simulink library "mobileRoboticsLib"  (R2022b)
settings: Solver=VariableStepAuto  StartTime=0.0  StopTime=10.0  RelTol=1e-3
undefined symbols (not defined in the file or in its folder): DiscIntNeverNeededParam, X, Y, Z
libraries: sm_lib x67, nesl_utility x25, $bdroot x12
(part 1 of 4)
settings Model: Creator=scastro  LastModifiedBy=mejiasal
settings SolverCC: AlgebraicLoopSolver=TrustRegion
settings DataIOCC: ReturnWorkspaceOutputs=off
settings DebuggingCC: UnconnectedInputMsg=warning  UnconnectedOutputMsg=warning  UnconnectedLineMsg=warning  SFMachineParentedDataDiag=warning  ArithmeticOperatorsInVariantConditions=warning
settings ModelReferenceCC: EnableRefExpFcnMdlSchedulingChecks=on
settings SFSimCC: SimUseLocalCustomCode=off  CustomCodeUndefinedFunction=UseInterfaceOnly
settings RTWCC: RTWUseLocalCustomCode=off

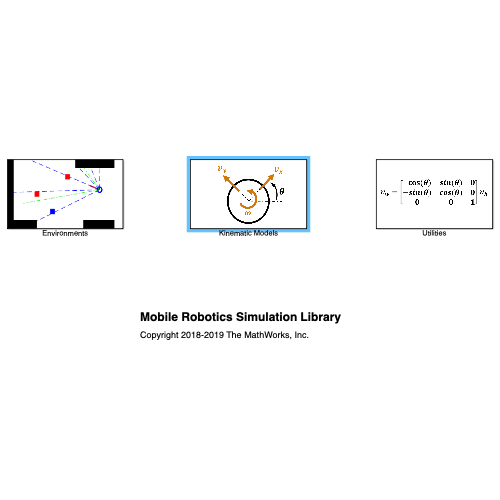
[thumbnail: Simulink's stored preview of the top-level diagram]
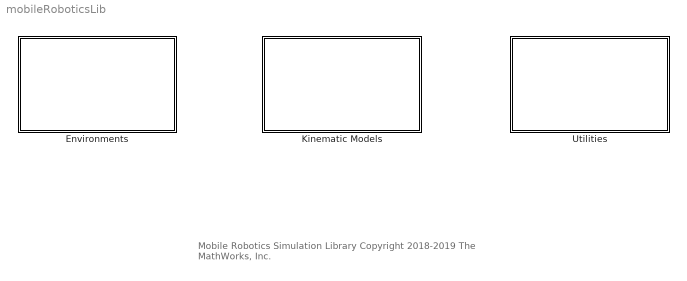
== system mobileRoboticsLib ==
  note: Mobile Robotics Simulation Library
      |
      | Copyright 2018-2019 The MathWorks, Inc.
  Environments : Subsystem
      mask Display: image('environments.PNG');
  Kinematic Models : Subsystem
      mask Display: image('kinematics.PNG')
  Utilities : Subsystem
      mask Display: image('mrsUtils.PNG');

== system mobileRoboticsLib/Environments ==
  Lidar Sensor : MATLABSystem  System=LidarSensor  sensorOffset=[ 0, 0 ]  scanAngles=[ -pi/4, 0, pi/4 ]  maxRange=5
      mask Type: LidarSensor
      mask Display:
      | disp(['Lidar' char(10) 'Sensor']);
      | port_label('input',1,'pose');
      | port_label('output',1,'ranges');
  Multi-Robot Environment : Subsystem  InitFcn=clear multiRobotVizWorld;  mask(Multi-Robot Environment){numRobots=3, mapName=, showWaypoints=off, showObjects=off, objectColors=[ 1, 0, 0; 0, 1, 0; 0, 0, 1 ], objectMarkers='s', showRobotIds=on, plotSensorLines=on}
      mask prompts: numRobots "Number of Robots"; mapName "Map Name"; showWaypoints "Accept Waypoints"; showObjects "Accept Objects"; objectColors "Object Colors"; objectMarkers "Object Markers"; showRobotIds "Show Robot IDs"; plotSensorLines "Plot Sensor Lines"
      mask help:
      | Displays map, waypoint, and object data for a multi-robot simulation.
      |
      | Use "Multi-Robot Visualizer" blocks to display individual robots in this environment.
      mask init:
      | % Configure visual tags
      | visualSub = [gcb '/Visuals'];
      | radiusBlocks = find_system(visualSub,'FollowLinks','on','LookUnderMasks','on','BlockType','From');
      | for idx = 1:numel(radiusBlocks)
      |     lh = get_param(radiusBlocks{idx},'LineHandles');
      |     delete_line(lh.Outport);
      | end
      | delete_block(radiusBlocks);
      | vecBlock = [visualSub '/Vector Concatenate'];
      | set_param(vecBlock,'NumInputs',num2str(numRobots));
      | for idx = 1:numRobots
      |     blkName = [visualSub '/From' num2str(idx)];
      |     blkPos = [0 30 200 50] + (idx-1)*[0 30 0 30];
      |     add_block('simulink/Signal Routing/From',blkName);
      |     set_param(blkName,'GotoTag',['slMultiRobotEnv_Visuals_' num2str(idx)]);
      |     set_param(blkName,'Position',blkPos);
      |     add_line(visualSub,['From' num2str(idx) '/1'],['Vector Concatenate/' num2str(idx)]);
      | end
      | 
      | % Configure pose tags
      | poseSub = [gcb '/Poses'];
      | poseBlocks = find_system(poseSub,'FollowLinks','on','LookUnderMasks','on','BlockType','From');
      | for idx = 1:numel(poseBlocks)
      |     lh = get_param(poseBlocks{idx},'LineHandles');
      |     delete_line(lh.Outport);
      | end
      | delete_block(poseBlocks);
      | vecBlock = [poseSub '/Vector Concatenate'];
      | set_param(vecBlock,'NumInputs',num2str(numRobots));
      | for idx = 1:numRobots
      |     blkName = [poseSub '/From' num2str(idx)];
      |     blkPos = [0 30 200 50] + (idx-1)*[0 30 0 30];
      |     add_block('simulink/Signal Routing/From',blkName);
      |     set_param(blkName,'GotoTag',['slMultiRobotEnv_Pose_' num2str(idx)]);
      |     set_param(blkName,'Position',blkPos);
      |     add_line(poseSub,['From' num2str(idx) '/1'],['Vector Concatenate/' num2str(idx)]);
      | end
      | 
      | % Configure range tags
      | rangeSub = [gcb '/Ranges'];
      | rangeBlocks = find_system(rangeSub,'FollowLinks','on','LookUnderMasks','on','BlockType','From');
      | for idx = 1:numel(rangeBlocks)
      |     lh = get_param(rangeBlocks{idx},'LineHandles');
      |     delete_line(lh.Outport);
      | end
      | delete_block(rangeBlocks);
      | vecBlock = [rangeSub '/Vector Concatenate'];
      | set_param(vecBlock,'NumInputs',num2str(numRobots));
      | for idx = 1:numRobots
      |     blkName = [rangeSub '/From' num2str(idx)];
      |     blkPos = [0 30 200 50] + (idx-1)*[0 30 0 30];
      |     add_block('simulink/Signal Routing/From',blkName);
      |     set_param(blkName,'GotoTag',['slMultiRobotEnv_Ranges_' num2str(idx)]);
      |     set_param(blkName,'Position',blkPos);
      |     add_line(rangeSub,['From' num2str(idx) '/1'],['Vector Concatenate/' num2str(idx)]);
      | end
      | 
      | % Initialize range sensor bus
      | internal.createRangeSensorBus;
      | 
      | % Configure object detector tags
      | objDetSub = [gcb '/ObjectDetectorParams'];
      | objDetBlocks = find_system(objDetSub,'FollowLinks','on','LookUnderMasks','on','BlockType','From');
      | for idx = 1:numel(objDetBlocks)
      |     lh = get_param(objDetBlocks{idx},'LineHandles');
      |     delete_line(lh.Outport);
      | end
      | delete_block(objDetBlocks);
      | vecBlock = [objDetSub '/Vector Concatenate'];
      | set_param(vecBlock,'NumInputs',num2str(numRobots));
      | for idx = 1:numRobots
      |     blkName = [objDetSub '/From' num2str(idx)];
      |     blkPos = [0 30 200 50] + (idx-1)*[0 30 0 30];
      |     add_block('simulink/Signal Routing/From',blkName);
      |     set_param(blkName,'GotoTag',['slMultiRobotEnv_ObjDet_' num2str(idx)]);
      |     set_param(blkName,'Position',blkPos);
      |     add_line(objDetSub,['From' num2str(idx) '/1'],['Vector Concatenate/' num2str(idx)]);
      | end
      | 
      | % Configure robot detector tags
      | robotDetSub = [gcb '/RobotDetectorParams'];
      | robotDetBlocks = find_system(robotDetSub,'FollowLinks','on','LookUnderMasks','on','BlockType','From');
      | for idx = 1:numel(robotDetBlocks)
      |     lh = get_param(robotDetBlocks{idx},'LineHandles');
      |     delete_line(lh.Outport);
      | end
      | delete_block(robotDetBlocks);
      | vecBlock = [robotDetSub '/Vector Concatenate'];
      | set_param(vecBlock,'NumInputs',num2str(numRobots));
      | for idx = 1:numRobots
      |     blkName = [robotDetSub '/From' num2str(idx)];
      |     blkPos = [0 30 200 50] + (idx-1)*[0 30 0 30];
      |     add_block('simulink/Signal Routing/From',blkName);
      |     set_param(blkName,'GotoTag',['slMultiRobotEnv_RobotDet_' num2str(idx)]);
      |     set_param(blkName,'Position',blkPos);
      |     add_line(robotDetSub,['From' num2str(idx) '/1'],['Vector Concatenate/' num2str(idx)]);
      | end
      | 
      | % Configure waypoints port
      | hasWaypointPort = ~isempty(find_system(gcb,'FollowLinks','on','LookUnderMasks','on','BlockType','Inport','Name','waypoints'));
      | if ~showWaypoints & hasWaypointPort
      |     replace_block(gcb,'FollowLinks','on','Name','waypoints','built-in/Ground','noprompt');
      | elseif showWaypoints & ~hasWaypointPort
      |     replace_block(gcb,'FollowLinks','on','Name','waypoints','built-in/Inport','noprompt'); 
      | end
      |  
      | % Configure objects port
      | hasObjectPort = ~isempty(find_system(gcb,'FollowLinks','on','LookUnderMasks','on','BlockType','Inport','Name','objects'));
      | if ~showObjects & hasObjectPort
      |     replace_block(gcb,'FollowLinks','on','Name','objects','built-in/Ground','noprompt');
      | elseif showObjects & ~hasObjectPort
      |     replace_block(gcb,'FollowLinks','on','Name','objects','built-in/Inport','noprompt');  
      | end
      | 
      | % Ensure the waypoints and objects ports are organized correctly
      | if strcmp(get_param([gcb '/waypoints'],'BlockType'),'Inport')
      |     set_param([gcb '/waypoints'],'Port','1');
      | end
      mask Help: web('matlab: edit mrsDocMultiRobotEnv')
      mask Callback showObjects:
      | mask = Simulink.Mask.get(gcb);
      | showObjects = get_param(gcb,'showObjects');
      | 
      | % Enable and disable parameters
      | indices = [find(strcmp({mask.Parameters.Name},'objectColors'));
      |            find(strcmp({mask.Parameters.Name},'objectMarkers'))];
      | 
      | for idx = 1:numel(indices)
      |     mask.Parameters(indices(idx)).Visible = showObjects;
      | end
      mask Display: fprintf('Multi-Robot\nEnvironment')
  Multi-Robot Lidar Sensor : Subsystem  mask(Multi-Robot Lidar Sensor){robotIdx=1, mapName=, sensorOffset=[0,0], scanAngles=[-pi/4 0 pi/4], maxRange=5}
      mask prompts: robotIdx "Robot Index"; mapName "Map Name"; sensorOffset "Sensor offset (x,y) [m]"; scanAngles "Scan angles [rad]"; maxRange "Maximum Range [m]"
      mask help: 2D lidar sensor simulation for multi-robot environment.
      mask init:
      | % Find number of robots 
      | mrEnvBlks = find_system(bdroot,'FollowLinks','on','LookUnderMasks','on','MaskType','Multi-Robot Environment');
      | mrEnvBlk = mrEnvBlks{1};
      | if isempty(mrEnvBlk)
      |     error('No Multi-Robot Environment found in model.')
      | end
      | numRobots = evalin('base',get_param(mrEnvBlk,'numRobots'));
      | 
      | % Configure pose tags
      | poseSub = [gcb '/Poses'];
      | poseBlocks = find_system(poseSub,'FollowLinks','on','LookUnderMasks','on','BlockType','From');
      | for idx = 1:numel(poseBlocks)
      |     lh = get_param(poseBlocks{idx},'LineHandles');
      |     delete_line(lh.Outport);
      | end
      | delete_block(poseBlocks);
      | vecBlock = [poseSub '/Vector Concatenate'];
      | set_param(vecBlock,'NumInputs',num2str(numRobots));
      | for idx = 1:numRobots
      |     blkName = [poseSub '/From' num2str(idx)];
      |     blkPos = [0 30 200 50] + (idx-1)*[0 30 0 30];
      |     add_block('simulink/Signal Routing/From',blkName);
      |     set_param(blkName,'GotoTag',['slMultiRobotEnv_Pose_' num2str(idx)]);
      |     set_param(blkName,'Position',blkPos);
      |     add_line(poseSub,['From' num2str(idx) '/1'],['Vector Concatenate/' num2str(idx)]);
      | end
      | 
      | % Configure visual tags
      | visualSub = [gcb '/Visuals'];
      | visualBlocks = find_system(visualSub,'FollowLinks','on','LookUnderMasks','on','BlockType','From');
      | for idx = 1:numel(visualBlocks)
      |     lh = get_param(visualBlocks{idx},'LineHandles');
      |     delete_line(lh.Outport);
      | end
      | delete_block(visualBlocks);
      | vecBlock = [visualSub '/Vector Concatenate'];
      | set_param(vecBlock,'NumInputs',num2str(numRobots));
      | for idx = 1:numRobots
      |     blkName = [visualSub '/From' num2str(idx)];
      |     blkPos = [0 30 200 50] + (idx-1)*[0 30 0 30];
      |     add_block('simulink/Signal Routing/From',blkName);
      |     set_param(blkName,'GotoTag',['slMultiRobotEnv_Visuals_' num2str(idx)]);
      |     set_param(blkName,'Position',blkPos);
      |     add_line(visualSub,['From' num2str(idx) '/1'],['Vector Concatenate/' num2str(idx)]);
      | end
      mask Help: web('matlab: edit mrsDocLidarSensor')
      mask Callback mapName:
      | % Update the map in the Robot Detector system object inside the mask
      | mapName = get_param(gcb,'mapName');
      | blkName = [gcb '/Multi-Robot Lidar Sensor'];
      | set_param(blkName,'mapName',mapName);
      mask Display:
      | idx = get_param(gcb,'robotIdx');
      | fprintf(['Multi Robot\nLidar ' idx])
  Multi-Robot Visualizer : Subsystem  mask(Multi-Robot Visualizer){idx=1, radius=0.25, robotColor=[0 0 1], showTraj=on, hasLidar=off, sensorOffset=[0,0], scanAngles=[-pi/4 0 pi/4], maxNumScans=0, hasObjDetector=off, objDetectorOffset=[0,0], objDetectorAngle=0, objDetectorFOV=pi/3, objDetectorMaxRange=5, hasRobotDetector=off, robotDetectorOffset=[0,0], robotDetectorAngle=0, robotDetectorFOV=pi/3, robotDetectorMaxRange=5, robotDetectorNumDetections=0}
      mask prompts: idx "Robot Index"; radius "Robot Radius [m]"; robotColor "Robot Color"; showTraj "Show Trajectory"; hasLidar "Accept Lidar"; sensorOffset "Lidar sensor offset (x,y) [m]"; scanAngles "Scan angles [rad]"; maxNumScans "Maximum number of scans"; hasObjDetector "Accept Object Detector"; objDetectorOffset "Object detector offset (x,y) [m]"; objDetectorAngle "Object detector angle [rad]"; objDetectorFOV "Object detector field of view [rad]"; objDetectorMaxRange "Object detector maximum range [m]"; hasRobotDetector "Accept Robot Detector"; robotDetectorOffset "Robot detector offset (x,y) [m]"; robotDetectorAngle "Robot detector angle [rad]"; robotDetectorFOV "Robot detector field of view [rad]"; robotDetectorMaxRange "Robot detector maximum range [m]"; robotDetectorNumDetections "Maximum number of detections"
      mask help:
      | Supply the pose and (optionally) lidar ranges for a single robot in a multi-robot setup.
      |
      | These blocks require a "Multi-Robot Environment" block to exist in the model.
      mask init:
      | % Configure ranges port
      | if ~hasLidar & ~isempty(find_system(gcb,'FollowLinks','on','LookUnderMasks','on','BlockType','Inport','Name','ranges'))
      |     replace_block(gcb,'FollowLinks','on','Name','ranges','built-in/Ground','noprompt');
      | elseif hasLidar & isempty(find_system(gcb,'FollowLinks','on','LookUnderMasks','on','BlockType','Inport','Name','ranges'))
      |     replace_block(gcb,'FollowLinks','on','Name','ranges','built-in/Inport','noprompt');  
      | end
      | 
      | % Set up the Goto tag numbers
      | set_param([gcb '/Goto_Visuals'],'GotoTag',['slMultiRobotEnv_Visuals_' num2str(idx)]);
      | set_param([gcb '/Goto_Pose'],'GotoTag',['slMultiRobotEnv_Pose_' num2str(idx)]);
      | set_param([gcb '/Goto_Ranges'],'GotoTag',['slMultiRobotEnv_Ranges_' num2str(idx)]);
      | set_param([gcb '/Goto_ObjDetector'],'GotoTag',['slMultiRobotEnv_ObjDet_' num2str(idx)]);
      | set_param([gcb '/Goto_RobotDetector'],'GotoTag',['slMultiRobotEnv_RobotDet_' num2str(idx)]);
      | 
      | % Get the maximum number of scans
      | maxNumScans = internal.getMaxNumScans;
      | 
      | % Initialize range sensor bus
      | internal.createRangeSensorBus;
      mask Help: web('matlab: edit mrsDocMultiRobotEnv')
      mask Callback hasLidar:
      | mask = Simulink.Mask.get(gcb);
      | hasLidar = get_param(gcb,'hasLidar');
      | 
      | % Enable and disable parameters
      | indices = [find(strcmp({mask.Parameters.Name},'sensorOffset'));
      |            find(strcmp({mask.Parameters.Name},'scanAngles'))];
      | 
      | for idx = 1:numel(indices)
      |     mask.Parameters(indices(idx)).Visible = hasLidar;
      | end
      mask Callback hasObjDetector:
      | mask = Simulink.Mask.get(gcb);
      | hasObjDetector = get_param(gcb,'hasObjDetector');
      | 
      | indices = [find(strcmp({mask.Parameters.Name},'objDetectorOffset'));
      |            find(strcmp({mask.Parameters.Name},'objDetectorAngle'));
      |            find(strcmp({mask.Parameters.Name},'objDetectorFOV'));
      |            find(strcmp({mask.Parameters.Name},'objDetectorMaxRange'))];
      | 
      | for idx = 1:numel(indices)
      |     mask.Parameters(indices(idx)).Visible = hasObjDetector;
      | end
      mask Callback hasRobotDetector:
      | mask = Simulink.Mask.get(gcb);
      | hasObjDetector = get_param(gcb,'hasRobotDetector');
      | 
      | indices = [find(strcmp({mask.Parameters.Name},'robotDetectorOffset'));
      |            find(strcmp({mask.Parameters.Name},'robotDetectorAngle'));
      |            find(strcmp({mask.Parameters.Name},'robotDetectorFOV'));
      |            find(strcmp({mask.Parameters.Name},'robotDetectorMaxRange'))];
      | 
      | for idx = 1:numel(indices)
      |     mask.Parameters(indices(idx)).Visible = hasObjDetector;
      | end
      mask DialogControl Container4 Prompt: Robot
      mask DialogControl Container6 Prompt: Sensors
      mask Display:
      | idx = get_param(gcb,'idx');
      | fprintf(['Robot ' idx '\n Visualizer'])
  Object Detector : MATLABSystem  System=ObjectDetector  sensorOffset=[ 0, 0 ]  sensorAngle=0  fieldOfView=pi/3  maxRange=5  maxDetections=3  sampleTime=0.1
      mask Type: ObjectDetector
      mask Display:
      | disp(['Object' char(10) 'Detector']);
      | port_label('input',1,'pose');
      | port_label('input',2,'objects');
      | port_label('output',1,'detections');
  Robot Detector : Subsystem  mask(Robot Detector){mapName=map, robotIdx=4, sensorOffset=[0,0], sensorAngle=0, sensorFOV=pi/3, maxRange=5, maxDetections=3, sampleTime=0.1}
      mask prompts: mapName "Map Name"; robotIdx "Robot Index"; sensorOffset "Sensor offset (x,y) [m]"; sensorAngle "Sensor angle [rad]"; sensorFOV "Sensor field of view [rad]"; maxRange "Maximum range [rad]"; maxDetections "Maximum number of detections"; sampleTime "Sample Time"
      mask help: Robot Detector Simulator
      mask init:
      | % Find number of robots 
      | mrEnvBlks = find_system(bdroot,'FollowLinks','on','LookUnderMasks','on','MaskType','Multi-Robot Environment');
      | mrEnvBlk = mrEnvBlks{1};
      | if isempty(mrEnvBlk)
      |     error('No Multi-Robot Environment found in model.')
      | end
      | numRobots = evalin('base',get_param(mrEnvBlk,'numRobots'));
      | 
      | % Configure pose tags
      | poseSub = [gcb '/Poses'];
      | poseBlocks = find_system(poseSub,'FollowLinks','on','LookUnderMasks','on','BlockType','From');
      | for idx = 1:numel(poseBlocks)
      |     lh = get_param(poseBlocks{idx},'LineHandles');
      |     delete_line(lh.Outport);
      | end
      | delete_block(poseBlocks);
      | vecBlock = [poseSub '/Vector Concatenate'];
      | set_param(vecBlock,'NumInputs',num2str(numRobots));
      | for idx = 1:numRobots
      |     blkName = [poseSub '/From' num2str(idx)];
      |     blkPos = [0 30 200 50] + (idx-1)*[0 30 0 30];
      |     add_block('simulink/Signal Routing/From',blkName);
      |     set_param(blkName,'GotoTag',['slMultiRobotEnv_Pose_' num2str(idx)]);
      |     set_param(blkName,'Position',blkPos);
      |     add_line(poseSub,['From' num2str(idx) '/1'],['Vector Concatenate/' num2str(idx)]);
      | end
      mask Help: web('matlab: edit mrsDocRobotDetector')
      mask Callback mapName:
      | % Update the map in the Robot Detector system object inside the mask
      | mapName = get_param(gcb,'mapName');
      | blkName = [gcb '/Robot Detector'];
      | set_param(blkName,'mapName',mapName);
      mask Display:
      | idx = get_param(gcb,'robotIdx');
      | fprintf(['Robot ' idx '\n Detector'])
  Robot Visualizer : MATLABSystem  System=Visualizer2D  robotRadius=0  showTrajectory=on  hasWaypoints=off  hasLidar=off  sensorOffset=[ 0, 0 ]  scanAngles=[ -pi/4, 0, pi/4 ]  hasObjDetector=on  objDetectorOffset=[ 0, 0 ]  objDetectorAngle=0  objDetectorFOV=pi/4  objDetectorMaxRange=5  objectColors=[ 1, 0, 0; 0, 1, 0; 0, 0, 1 ]  objectMarkers=s
      mask Type: Visualizer2D
      mask Display:
      | disp(['Robot' char(10) 'Visualizer']);
      | port_label('input',1,'pose');
      | port_label('input',2,'objects');

== system mobileRoboticsLib/Kinematic Models ==
  Differential Drive : Subsystem
      mask Display: image('diffDriveIcon.PNG')
  Four-Wheel Mecanum : Subsystem
      mask Display: image('mecanumIcon.PNG')
  Four-Wheel Steering : Subsystem
      mask Display: image('fourWheelSteerIcon.PNG')
  Generic Omniwheel : Subsystem
      mask Display: image('genericOmniIcon.png')
  Triple Omniwheel : Subsystem
      mask Display: image('tripleOmniIcon.PNG')

== system mobileRoboticsLib/Utilities ==
  Assign to Maximum Size : MATLAB Function  TreatAsAtomicUnit=on  mask{maxLength=25}
      mask prompts: maxLength "Maximum Length"
  Body to World Velocity : Subsystem  mask(Body to World Velocity){}
      mask help:
      | Converts a 2D velocity input [vx;vy;w] from body (vehicle) coordinates to world (global) coordinates.
      |
      | vx = Linear velocity in x-direction (longitudinal)
      | vy = Linear velocity in y-direction (lateral)
      | w = Angular velocity (about z-axis)
  Generic Vehicle Simulation : Subsystem  mask(Generic Vehicle Simulation){initX=2, initY=3, initAngle=0, Ts=0.05}
      mask prompts: initX "Initial X Position [m]"; initY "Initial Y Position [m]"; initAngle "Initial Angle (theta) [rad]"; Ts "Sample Time"
      mask help:
      | Simulates the kinematics of a generic vehicle, from a specified initial pose.
      |
      | Input: Body velocities [vx; vy; w], in m/s, m/s, and rad/s
      |
      | Output: Pose [x; y; theta], in m, m, and rad
      |
      | Set the Sample Time parameter to 0 for continuous-time simulation, or a positive number for discrete-time simulation.
      mask Callback Ts:
      | Ts = evalin('base',get_param(gcb,'Ts'));
      | blk = [gcb '/Velocity Integrator'];
      | if Ts > 0
      |     set_param(blk,'OverrideUsingVariant','mode==2');
      | else
      |     set_param(blk,'OverrideUsingVariant','mode==1');
      | end
  World to Body Velocity : Subsystem  mask(World to Body Velocity){}
      mask help:
      | Converts a 2D velocity input [vx;vy;w] from world (global) coordinates to body (vehicle) coordinates.
      |
      | vx = Linear velocity in x-direction (longitudinal)
      | vy = Linear velocity in y-direction (lateral)
      | w = Angular velocity (about z-axis)

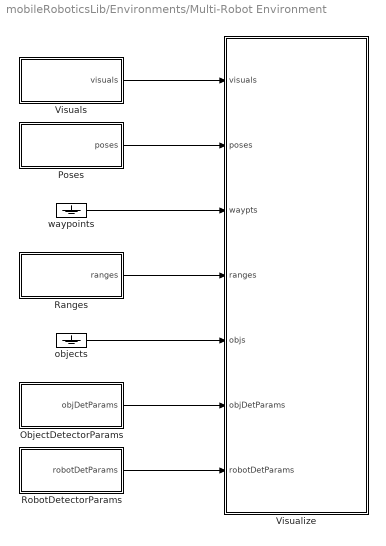
== system mobileRoboticsLib/Environments/Multi-Robot Environment ==
  ObjectDetectorParams : Subsystem
  Poses : Subsystem
  Ranges : Subsystem
  RobotDetectorParams : Subsystem
  Visualize : MATLAB Function  TreatAsAtomicUnit=on
  Visuals : Subsystem
  objects : Ground
  waypoints : Ground
  wires:
  RobotDetectorParams/1(robotDetParams) -> Visualize/7(robotDetParams)
  ObjectDetectorParams/1(objDetParams) -> Visualize/6(objDetParams)
  Visuals/1(visuals) -> Visualize/1(visuals)
  Poses/1(poses) -> Visualize/2(poses)
  Ranges/1(ranges) -> Visualize/4(ranges)
  waypoints/1 -> Visualize/3(waypts)
  objects/1 -> Visualize/5(objs)

== system mobileRoboticsLib/Environments/Multi-Robot Lidar Sensor ==
  Multi-Robot Lidar Sensor : MATLABSystem  System=MultiRobotLidarSensor  sensorOffset=sensorOffset  scanAngles=scanAngles  maxRange=maxRange  robotIdx=robotIdx  robotRadii=-1
      mask Type: MultiRobotLidarSensor
      mask Display:
      | disp(['Multi-Robot' char(10) 'Lidar 1']);
      | port_label('output',1,'ranges');
  Poses : Subsystem
  Visuals : Subsystem
  ranges : Outport  VectorParamsAs1DForOutWhenUnconnected=off
  wires:
  Poses/1(poses) -> Multi-Robot Lidar Sensor/1
  Multi-Robot Lidar Sensor/1 -> ranges/1
  Visuals/1(visuals) -> Multi-Robot Lidar Sensor/2

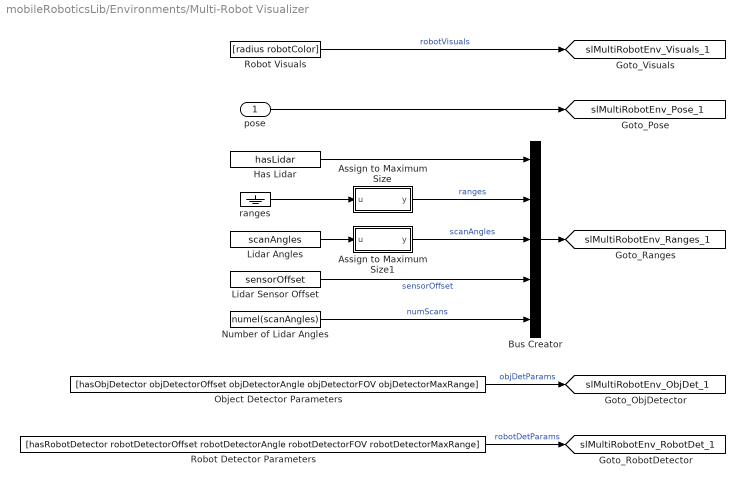
== system mobileRoboticsLib/Environments/Multi-Robot Visualizer ==
  pose : Inport
  Assign to Maximum Size : MATLAB Function  TreatAsAtomicUnit=on  mask{maxLength=maxNumScans}
      mask prompts: maxLength "Maximum Length"
  Assign to Maximum Size1 : MATLAB Function  TreatAsAtomicUnit=on  mask{maxLength=maxNumScans}
      mask prompts: maxLength "Maximum Length"
  Bus Creator : BusCreator  Inputs=5  OutDataTypeStr=Bus: slbus_MultiRobotRangeSensor  NonVirtualBus=on
      settings: InheritFromInputs=off
  Has Lidar : Constant  Value=hasLidar  OutDataTypeStr=boolean
  Lidar Angles : Constant  Value=scanAngles
  Lidar Sensor Offset : Constant  Value=sensorOffset
  Number of Lidar Angles : Constant  Value=numel(scanAngles)
  Object Detector Parameters : Constant  Value=[hasObjDetector objDetectorOffset objDetectorAngle objDetectorFOV objDetectorMaxRange]
  Robot Detector Parameters : Constant  Value=[hasRobotDetector robotDetectorOffset robotDetectorAngle robotDetectorFOV robotDetectorMaxRange]
  Robot Visuals : Constant  Value=[radius robotColor]
  ranges : Ground
  tag scope: slMultiRobotEnv_ObjDet_1=global, slMultiRobotEnv_Pose_1=global, slMultiRobotEnv_Ranges_1=global, slMultiRobotEnv_RobotDet_1=global, slMultiRobotEnv_Visuals_1=global
  wires:
  ranges/1 -> Assign to Maximum Size/1(u)
  pose/1 -> [slMultiRobotEnv_Pose_1]
  Bus Creator/1 -> [slMultiRobotEnv_Ranges_1]
  Lidar Sensor Offset/1 -> Bus Creator/4  "sensorOffset"
  Assign to Maximum Size/1(y) -> Bus Creator/2  "ranges"
  Lidar Angles/1 -> Assign to Maximum Size1/1(u)
  Assign to Maximum Size1/1(y) -> Bus Creator/3  "scanAngles"
  Number of Lidar Angles/1 -> Bus Creator/5  "numScans"
  Robot Visuals/1 -> [slMultiRobotEnv_Visuals_1]  "robotVisuals"
  Object Detector Parameters/1 -> [slMultiRobotEnv_ObjDet_1]  "objDetParams"
  Robot Detector Parameters/1 -> [slMultiRobotEnv_RobotDet_1]  "robotDetParams"
  Has Lidar/1 -> Bus Creator/1

== system mobileRoboticsLib/Environments/Robot Detector ==
  Poses : Subsystem
  Robot Detector : MATLABSystem  System=RobotDetector  mapName=map  robotIdx=robotIdx  sensorOffset=sensorOffset  sensorAngle=sensorAngle  fieldOfView=sensorFOV  maxRange=maxRange  maxDetections=maxDetections  sampleTime=sampleTime
      mask Type: RobotDetector
      mask Display:
      | disp(['Robot 4' char(10) 'Detector']);
      | port_label('output',1,'detections');
  detections : Outport  VectorParamsAs1DForOutWhenUnconnected=off
  wires:
  Robot Detector/1 -> detections/1
  Poses/1(poses) -> Robot Detector/1

== system mobileRoboticsLib/Kinematic Models/Differential Drive ==
  Differential Drive (Simscape Multibody Model) : Subsystem  mask(Differential Drive (Simscape Multibody Model)){wheelRadius=0.1, wheelBase=0.5, wheelThickness=0.025, chassisThickness=0.05, initX=0, initY=0, initAngle=0, timeConstant=0.05, wheelMass=0.1, chassisMass=1, wheelColor=[0.25 0.25 0.25], chassisColor=[0.8 0 0]}
      mask prompts: wheelRadius "Wheel Radius [m]"; wheelBase "Wheelbase [m]"; wheelThickness "Wheel Thickness [m]"; chassisThickness "Chassis Thickness [m]"; initX "Initial X Position [m]"; initY "Initial Y Position [m]"; initAngle "Initial Angle [rad]"; timeConstant "Motion Time Constant [s]"; wheelMass "Wheel Mass [kg]"; chassisMass "Chassis Mass [kg]"; wheelColor "Wheel Color"; chassisColor "Chassis Color"
      mask help:
      | Kinematics-only (motion actuated) Simscape Multibody Model of a differential drive vehicle.
      |
      | Inputs:
      | Left and right wheel speeds [wL; wR], in rad/s
      | Pose [x; y; theta], in m, m, and rad/s, respectively
      |
      | Connection Ports:
      | R: Reference frame at center of vehicle
      | G: Ground/world location
      mask Help: web('matlab:edit mrsDocDifferentialDrive')
      mask DialogControl KinContainer Prompt: Kinematics
      mask DialogControl DynamicsContainer Prompt: Dynamics
      mask DialogControl AppearanceContainer Prompt: Appearance
  Differential Drive Forward Kinematics : Subsystem  mask(Differential Drive Forward Kinematics){wheelRadius=0.1, wheelBase=0.5}
      mask prompts: wheelRadius "Wheel Radius [m]"; wheelBase "Wheelbase [m]"
      mask help:
      | Calculates the forward kinematics for a differential drive vehicle.
      |
      | Input: [wL; wR], the left and right wheel speeds (rad/s)
      |
      | Output: [v; w], the linear (m/s) and angular (rad/s) velocities of the vehicle
      mask Help: web('matlab:edit mrsDocDifferentialDrive')
  Differential Drive Inverse Kinematics : Subsystem  mask(Differential Drive Inverse Kinematics){wheelRadius=0.1, wheelBase=0.5}
      mask prompts: wheelRadius "Wheel Radius [m]"; wheelBase "Wheelbase [m]"
      mask help:
      | Calculates the forward kinematics for a differential drive vehicle.
      |
      | Input: [v; w], the linear (m/s) and angular (rad/s) velocities of the vehicle
      |
      | Output: [wL; wR], the left and right wheel speeds (rad/s)
      mask Help: web('matlab:edit mrsDocDifferentialDrive')
  Differential Drive Simulation : Subsystem  mask(Differential Drive Simulation){wheelRadius=0.1, wheelBase=0.5, initX=0, initY=0, initAngle=0, Ts=0.05}
      mask prompts: wheelRadius "Wheel Radius [m]"; wheelBase "Wheelbase [m]"; initX "Initial X Position [m]"; initY "Initial Y Position [m]"; initAngle "Initial Angle [rad]"; Ts "Sample Time"
      mask help:
      | Simulates the kinematics of a differential drive vehicle from a specified initial pose.
      |
      | Input: Left and right wheel speeds [wL; wR], in rad/s
      |
      | Output: Pose [x; y; theta], in m, m, and rad
      |
      | Set the Sample Time parameter to 0 for continuous-time simulation, or a positive number for discrete-time simulation.
      mask Help: web('matlab:edit mrsDocDifferentialDrive')
      mask Callback Ts:
      | Ts = evalin('base',get_param(gcb,'Ts'));
      | blk = [gcb '/Generic Robot Simulation/Velocity Integrator'];
      | if Ts > 0
      |     set_param(blk,'OverrideUsingVariant','mode==2');
      | else
      |     set_param(blk,'OverrideUsingVariant','mode==1');
      | end

== system mobileRoboticsLib/Kinematic Models/Four-Wheel Mecanum ==
  Four-Wheel Mecanum (Simscape Multibody Model) : Subsystem  mask(Four-Wheel Mecanum (Simscape Multibody Model)){wheelRadius=0.1, wheelBase=0.4, wheelTrack=0.5, wheelThickness=0.025, chassisThickness=0.05, initX=0, initY=0, initAngle=0, timeConstant=0.05, wheelMass=0.1, chassisMass=1, wheelColor=[0.25 0.25 0.25], chassisColor=[0.8 0 0]}
      mask prompts: wheelRadius "Wheel Radius [m]"; wheelBase "Wheelbase [m]"; wheelTrack "Track [m]"; wheelThickness "Wheel Thickness [m]"; chassisThickness "Chassis Thickness [m]"; initX "Initial X Position [m]"; initY "Initial Y Position [m]"; initAngle "Initial Angle [rad]"; timeConstant "Motion Time Constant [s]"; wheelMass "Wheel Mass [kg]"; chassisMass "Chassis Mass [kg]"; wheelColor "Wheel Color"; chassisColor "Chassis Color"
      mask help:
      | Kinematics-only (motion actuated) Simscape Multibody Model of a four-wheeled vehicle with Mecanum wheels.
      |
      | Inputs:
      | Wheel speeds [w1; w2; w3; w4] (rad/s)
      | Pose [x; y; theta], in m, m, and rad/s, respectively
      |
      | Connection Ports:
      | R: Reference frame at center of vehicle
      | G: Ground/world location
      mask Help: web('matlab:edit mrsDocFourWheelMecanum')
      mask DialogControl KinContainer Prompt: Kinematics
      mask DialogControl DynamicsContainer Prompt: Dynamics
      mask DialogControl AppearanceContainer Prompt: Appearance
  Four-Wheel Mecanum Forward Kinematics : Subsystem  mask(Four-Wheel Mecanum Forward Kinematics){wheelRadius=0.1, wheelBase=0.4, wheelTrack=0.5}
      mask prompts: wheelRadius "Wheel Radius [m]"; wheelBase "Wheelbase [m]"; wheelTrack "Track [m]"
      mask help:
      | Calculates the forward kinematics for a four-wheeled vehicle with Mecanum wheels.
      |
      | Input: Wheel speeds [w1; w2; w3; w4] (rad/s)
      |
      | Output: Vehicle velocities [vx; vy; w] in body coordinates (m/s, m/s, and rad/s)
      mask Help: web('matlab:edit mrsDocFourWheelMecanum')
  Four-Wheel Mecanum Inverse Kinematics : Subsystem  mask(Four-Wheel Mecanum Inverse Kinematics){wheelRadius=0.1, wheelBase=0.4, wheelTrack=0.5}
      mask prompts: wheelRadius "Wheel Radius [m]"; wheelBase "Wheelbase [m]"; wheelTrack "Track [m]"
      mask help:
      | Calculates the inverse kinematics for a four-wheeled vehicle with Mecanum wheels.
      |
      | Input: Vehicle velocities [vx; vy; w] in body coordinates (m/s, m/s, and rad/s)
      |
      | Output: Wheel speeds [w1; w2; w3; w4] (rad/s)
      mask Help: web('matlab:edit mrsDocFourWheelMecanum')
  Four-Wheel Mecanum Simulation : Subsystem  mask(Four-Wheel Mecanum Simulation){wheelRadius=0.1, wheelBase=0.4, wheelTrack=0.5, initX=0, initY=0, initAngle=0, Ts=0.05}
      mask prompts: wheelRadius "Wheel Radius [m]"; wheelBase "Wheelbase [m]"; wheelTrack "Track [m]"; initX "Initial X Position [m]"; initY "Initial Y Position [m]"; initAngle "Initial Angle [rad]"; Ts "Sample Time"
      mask help:
      | Simulates the kinematics of a four-wheeled vehicle with Mecanum wheels, from a specified initial pose.
      |
      | Input: Wheel speeds [w1; w2; w3; w4] (rad/s)
      |
      | Output: Pose [x; y; theta], in m, m, and rad
      |
      | Set the Sample Time parameter to 0 for continuous-time simulation, or a positive number for discrete-time simulation.
      mask Help: web('matlab:edit mrsDocFourWheelMecanum')
      mask Callback Ts:
      | Ts = evalin('base',get_param(gcb,'Ts'));
      | blk = [gcb '/Generic Robot Simulation/Velocity Integrator'];
      | if Ts > 0
      |     set_param(blk,'OverrideUsingVariant','mode==2');
      | else
      |     set_param(blk,'OverrideUsingVariant','mode==1');
      | end

== system mobileRoboticsLib/Kinematic Models/Four-Wheel Steering ==
  Four-Wheel Steering (Simscape Multibody Model) : Subsystem  mask(Four-Wheel Steering (Simscape Multibody Model)){wheelRadius=0.1, wheelBase=0.3, frontLen=0.25, rearLen=0.25, wheelThickness=0.025, chassisThickness=0.05, initX=0, initY=0, initAngle=0, timeConstant=0.05, wheelMass=0.1, chassisMass=1, wheelColor=[0.25 0.25 0.25], chassisColor=[0.8 0 0]}
      mask prompts: wheelRadius "Wheel Radius [m]"; wheelBase "Wheelbase [m]"; frontLen "CG to Front Wheel Distance [m]"; rearLen "CG to Rear Wheel Distance [m]"; wheelThickness "Wheel Thickness [m]"; chassisThickness "Chassis Thickness [m]"; initX "Initial X Position [m]"; initY "Initial Y Position [m]"; initAngle "Initial Angle [rad]"; timeConstant "Motion Time Constant [s]"; wheelMass "Wheel Mass [kg]"; chassisMass "Chassis Mass [kg]"; wheelColor "Wheel Color"; chassisColor "Chassis Color"
      mask help:
      | Kinematics-only (motion actuated) Simscape Multibody Model of a four-wheeled vehicle with front and rear drive and steering.
      |
      | Input:
      | Wheel speeds [wf; wr] (rad/s)
      | Steer angles [phif; phir] (rad)
      | Pose [x; y; theta], in m, m, and rad/s, respectively
      |
      | Connection Ports:
      | R: Reference frame at center of vehicle
      | G: Ground/world location
      mask Help: web('matlab:edit mrsDocFourWheelSteer')
      mask DialogControl KinContainer Prompt: Kinematics
      mask DialogControl DynamicsContainer Prompt: Dynamics
      mask DialogControl AppearanceContainer Prompt: Appearance
  Four-Wheel Steering Forward Kinematics : Subsystem  mask(Four-Wheel Steering Forward Kinematics){wheelRadius=0.1, frontWheelDist=0.25, rearWheelDist=0.25}
      mask prompts: wheelRadius "Wheel Radius [m]"; frontWheelDist "CG to Front Wheel Distance [m]"; rearWheelDist "CG to Rear Wheel Distance [m]"
      mask help:
      | Calculates the forward kinematics for a four-wheeled vehicle with front and rear drive and steering.
      |
      | Input:
      | Wheel speeds [wf; wr] (rad/s)
      | Steer angles [phif; phir] (rad)
      |
      | Output: Vehicle velocities [vx; vy; w] in body coordinates (m/s, m/s, and rad/s)
      mask Help: web('matlab:edit mrsDocFourWheelSteer')
  Four-Wheel Steering Inverse Kinematics : Subsystem  mask(Four-Wheel Steering Inverse Kinematics){wheelRadius=0.1, frontWheelDist=0.25, rearWheelDist=0.25, ikMode=Front Steering}
      mask prompts: wheelRadius "Wheel Radius [m]"; frontWheelDist "CG to Front Wheel Distance [m]"; rearWheelDist "CG to Rear Wheel Distance [m]"; ikMode "Inverse Kinematics Mode"
      mask help:
      | Calculates the inverse kinematics for a four-wheeled vehicle with front and rear drive and steering.
      |
      | Input:
      | Vehicle velocities [vx; vy; w] in body coordinates (m/s, m/s, and rad/s)
      | In Front Steering and Zero Sideslip mode, the velocity inputs used are forward and angular speed [vx;w]
      | In Parallel Steering mode, the velocity inputs used are forward and lateral speed [vx;vy]
      |
      | Output:
      | Wheel speeds [wf; wr] (rad/s)
      | Steer angles [phif; phir] (rad)
      mask init:
      | blk = [gcb '/Inverse Kinematics'];
      | varStr = ['mode==' num2str(ikMode)];
      | set_param(blk,'OverrideUsingVariant',varStr);
      mask Help: web('matlab:edit mrsDocFourWheelSteer')
      mask TypeOptions ikMode: Front Steering | Parallel Steering | Zero Sideslip
      mask Display:
      | text(0.5,0.9,get_param(gcb,'ikMode'), ...
      |      'horizontalAlignment','center');
  Four-Wheel Steering Simulation : Subsystem  mask(Four-Wheel Steering Simulation){wheelRadius=0.1, frontWheelDist=0.25, rearWheelDist=0.25, initX=0, initY=0, initAngle=0, Ts=0.05}
      mask prompts: wheelRadius "Wheel Radius [m]"; frontWheelDist "CG to Front Wheel Distance [m]"; rearWheelDist "CG to Rear Wheel Distance [m]"; initX "Initial X Position [m]"; initY "Initial Y Position [m]"; initAngle "Initial Angle [rad]"; Ts "Sample Time"
      mask help:
      | Simulates the kinematics of a four-wheeled vehicle with front and rear drive and steering, from a specified initial pose.
      |
      | Input:
      | Wheel speeds [wf; wr] (rad/s)
      | Steer angles [phif; phir] (rad)
      |
      | Output: Pose [x; y; theta], in m, m, and rad
      |
      | Set the Sample Time parameter to 0 for continuous-time simulation, or a positive number for discrete-time simulation.
      mask Help: web('matlab:edit mrsDocFourWheelSteer')
      mask Callback Ts:
      | Ts = evalin('base',get_param(gcb,'Ts'));
      | blk = [gcb '/Generic Robot Simulation/Velocity Integrator'];
      | if Ts > 0
      |     set_param(blk,'OverrideUsingVariant','mode==2');
      | else
      |     set_param(blk,'OverrideUsingVariant','mode==1');
      | end
  Four-Wheel Steering Simulation w/speed : $bdroot/Kinematic Models/Four-Wheel Steering/Four-Wheel Steering Simulation  wheelRadius=0.1  frontWheelDist=0.25  rearWheelDist=0.25  initX=0  initY=0  initAngle=0  Ts=0.05

== system mobileRoboticsLib/Kinematic Models/Generic Omniwheel ==
  Generic Omniwheel Forward Kinematics : Subsystem  mask(Generic Omniwheel Forward Kinematics){wheelRadius=0.1, wheelPositions=[1 1;-1 1;-1 -1;1 -1], wheelAngles=[0; pi/4; -pi/4; 0]}
      mask prompts: wheelRadius "Wheel Radius [m]"; wheelPositions "Wheel (X,Y) Positions [m]"; wheelAngles "Wheel Angles [rad]"
      mask help:
      | Calculates the forward kinematics for an N-wheeled vehicle with omniwheels.
      |
      | Input: Wheel speeds [w1; w2; ... ; wN] (rad/s)
      |
      | Output: Vehicle velocities [vx; vy; w] in body coordinates (m/s, m/s, and rad/s)
      mask Help: web('matlab:edit mrsDocGenericOmniwheel')
  "Generic Omniwheel Inverse Kinematics " : Subsystem  mask(Generic Omniwheel Inverse Kinematics){wheelRadius=0.1, wheelPositions=[1 1;-1 1;-1 -1;1 -1], wheelAngles=[0; pi/4; -pi/4; 0]}
      mask prompts: wheelRadius "Wheel Radius [m]"; wheelPositions "Wheel (X,Y) Positions [m]"; wheelAngles "Wheel Angles [rad]"
      mask help:
      | Calculates the inverse kinematics for an N-wheeled vehicle with omniwheels.
      |
      | Input: Vehicle velocities [vx; vy; w] in body coordinates (m/s, m/s, and rad/s)
      |
      | Output: Wheel speeds [w1; w2; ... ; wN] (rad/s)
      mask Help: web('matlab:edit mrsDocGenericOmniwheel')
  Generic Omniwheel Simulation : Subsystem  mask(Generic Omniwheel Simulation){wheelRadius=0.1, wheelPositions=[1 1;-1 1;-1 -1;1 -1], wheelAngles=[0; pi/4; -pi/4; 0], initX=0, initY=0, initAngle=0, Ts=0.05}
      mask prompts: wheelRadius "Wheel Radius [m]"; wheelPositions "Wheel (X,Y) Positions [m]"; wheelAngles "Wheel Angles [rad]"; initX "Initial X Position [m]"; initY "Initial Y Position [m]"; initAngle "Initial Angle [rad]"; Ts "Sample Time"
      mask help:
      | Simulates the kinematics of an N-wheeled vehicle with omniwheels, from a specified initial pose.
      |
      | Input: Wheel speeds [w1; w2; ... ; wN] (rad/s)
      |
      | Output: Pose [x; y; theta], in m, m, and rad
      |
      | Set the Sample Time parameter to 0 for continuous-time simulation, or a positive number for discrete-time simulation.
      mask Help: web('matlab:edit mrsDocGenericOmniwheel')
      mask Callback Ts:
      | Ts = evalin('base',get_param(gcb,'Ts'));
      | blk = [gcb '/Generic Robot Simulation/Velocity Integrator'];
      | if Ts > 0
      |     set_param(blk,'OverrideUsingVariant','mode==2');
      | else
      |     set_param(blk,'OverrideUsingVariant','mode==1');
      | end

== system mobileRoboticsLib/Kinematic Models/Triple Omniwheel ==
  Triple Omniwheel (Simscape Multibody Model) : Subsystem  mask(Triple Omniwheel (Simscape Multibody Model)){wheelRadius=0.1, robotRadius=0.25, wheelAngles=[0,2*pi/3,-2*pi/3], wheelThickness=0.025, chassisThickness=0.05, initX=2, initY=3, initAngle=0, timeConstant=0.05, wheelMass=0.1, chassisMass=1, wheelColor=[0.25 0.25 0.25], chassisColor=[0.8 0 0]}
      mask prompts: wheelRadius "Wheel Radius [m]"; robotRadius "Robot Radius [m]"; wheelAngles "Wheel Angles [rad]"; wheelThickness "Wheel Thickness [m]"; chassisThickness "Chassis Thickness [m]"; initX "Initial X Position [m]"; initY "Initial Y Position [m]"; initAngle "Initial Angle [rad]"; timeConstant "Motion Time Constant [s]"; wheelMass "Wheel Mass [kg]"; chassisMass "Chassis Mass [kg]"; wheelColor "Wheel Color"; chassisColor "Chassis Color"
      mask help:
      | Kinematics-only (motion actuated) Simscape Multibody Model of a three-wheeled vehicle with omniwheels.
      |
      | Inputs:
      | Wheel speeds [w1; w2; w3] (rad/s)
      | Pose [x; y; theta], in m, m, and rad/s, respectively
      |
      | Connection Ports:
      | R: Reference frame at center of vehicle
      | G: Ground/world location
      mask Help: web('matlab:edit mrsDocTripleOmniwheel')
      mask DialogControl KinContainer Prompt: Kinematics
      mask DialogControl DynamicsContainer Prompt: Dynamics
      mask DialogControl AppearanceContainer Prompt: Appearance
  Triple Omniwheel Forward Kinematics : Subsystem  mask(Triple Omniwheel Forward Kinematics){wheelRadius=0.1, robotRadius=0.25, wheelAngles=[0,2*pi/3,-2*pi/3]}
      mask prompts: wheelRadius "Wheel Radius [m]"; robotRadius "Robot Radius [m]"; wheelAngles "Wheel Angles [rad]"
      mask help:
      | Calculates the forward kinematics for a three-wheeled vehicle with omniwheels.
      |
      | Input: Wheel speeds [w1; w2; w3] (rad/s)
      |
      | Output: Vehicle velocities [vx; vy; w] in body coordinates (m/s, m/s, and rad/s)
      mask Help: web('matlab:edit mrsDocTripleOmniwheel')
  "Triple Omniwheel Inverse Kinematics " : Subsystem  mask(Triple Omniwheel Inverse Kinematics){wheelRadius=0.1, robotRadius=0.25, wheelAngles=[0,2*pi/3,-2*pi/3]}
      mask prompts: wheelRadius "Wheel Radius [m]"; robotRadius "Robot Radius [m]"; wheelAngles "Wheel Angles [rad]"
      mask help:
      | Calculates the inverse kinematics for a three-wheeled vehicle with omniwheels.
      |
      | Input: Vehicle velocities [vx; vy; w] in body coordinates (m/s, m/s, and rad/s)
      |
      | Output: Wheel speeds [w1; w2; w3] (rad/s)
      mask Help: web('matlab:edit mrsDocTripleOmniwheel')
  Triple Omniwheel Simulation : Subsystem  mask(Triple Omniwheel Simulation){wheelRadius=0.1, robotRadius=0.25, wheelAngles=[0,2*pi/3,-2*pi/3], initX=0, initY=0, initAngle=0, Ts=0.05}
      mask prompts: wheelRadius "Wheel Radius [m]"; robotRadius "Robot Radius [m]"; wheelAngles "Wheel Angles [rad]"; initX "Initial X Position [m]"; initY "Initial Y Position [m]"; initAngle "Initial Angle [rad]"; Ts "Sample Time"
      mask help:
      | Simulates the kinematics of a three-wheeled vehicle with omniwheels, from a specified initial pose.
      |
      | Input: Wheel speeds [w1; w2; w3] (rad/s)
      |
      | Output: Pose [x; y; theta], in m, m, and rad
      |
      | Set the Sample Time parameter to 0 for continuous-time simulation, or a positive number for discrete-time simulation.
      mask Help: web('matlab:edit mrsDocTripleOmniwheel')
      mask Callback Ts:
      | Ts = evalin('base',get_param(gcb,'Ts'));
      | blk = [gcb '/Generic Robot Simulation/Velocity Integrator'];
      | if Ts > 0
      |     set_param(blk,'OverrideUsingVariant','mode==2');
      | else
      |     set_param(blk,'OverrideUsingVariant','mode==1');
      | end

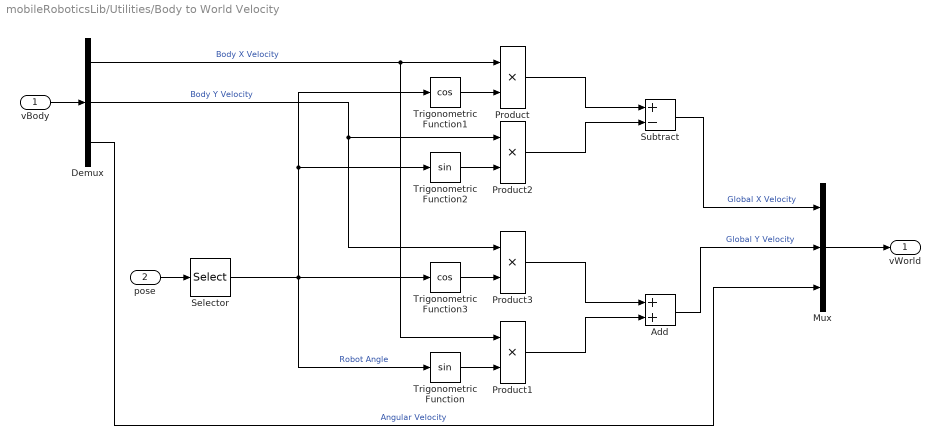
== system mobileRoboticsLib/Utilities/Body to World Velocity ==
  vBody : Inport
  pose : Inport  Port=2
  Add : Sum
  Demux : Demux  Outputs=3
  Mux : Mux  Inputs=3
  Product{,1..3} (4 alike) : Product
  Selector : Selector  InputPortWidth=3  IndexOptions=Index vector (dialog)  Indices=3  OutputSizes=1
  Subtract : Sum  Inputs=+-
  Trigonometric Function : Trigonometry
  Trigonometric Function1 : Trigonometry  Operator=cos
  Trigonometric Function2 : Trigonometry
  Trigonometric Function3 : Trigonometry  Operator=cos
  vWorld : Outport  VectorParamsAs1DForOutWhenUnconnected=off
  wires:
  pose/1 -> Selector/1
  Add/1 -> Mux/2  "Global Y Velocity"
  Product3/1 -> Add/1
  Trigonometric Function3/1 -> Product3/2
  Product2/1 -> Subtract/2
  Demux/2 -> Product2/1, Product3/1  "Body Y Velocity"
  Trigonometric Function2/1 -> Product2/2
  Subtract/1 -> Mux/1  "Global X Velocity"
  Selector/1 -> Trigonometric Function/1, Trigonometric Function1/1, Trigonometric Function2/1, Trigonometric Function3/1  "Robot Angle"
  Demux/1 -> Product/1, Product1/1  "Body X Velocity"
  Trigonometric Function1/1 -> Product/2
  Product/1 -> Subtract/1
  Product1/1 -> Add/2
  Trigonometric Function/1 -> Product1/2
  vBody/1 -> Demux/1
  Mux/1 -> vWorld/1
  Demux/3 -> Mux/3  "Angular Velocity"

== system mobileRoboticsLib/Utilities/Generic Vehicle Simulation ==
  bodySpd : Inport
  Body to Cartesian Velocity : $bdroot/Utilities/Body to World Velocity
  Demux1 : Demux  Outputs=3
  Mux : Mux  Inputs=3
  Velocity Integrator : Subsystem  Variant=on  VariantControlMode=label  VariantControl=Variant1  LabelModeActiveChoice=mode==2
  pose : Outport  VectorParamsAs1DForOutWhenUnconnected=off
  wires:
  bodySpd/1 -> Body to Cartesian Velocity/1
  Demux1/3 -> Velocity Integrator/3("w ")
  Demux1/2 -> Velocity Integrator/2("vy ")
  Demux1/1 -> Velocity Integrator/1("vx ")
  Body to Cartesian Velocity/1 -> Demux1/1
  Mux/1 -> pose/1, Body to Cartesian Velocity/2
  Velocity Integrator/1(" x") -> Mux/1
  Velocity Integrator/2(" y") -> Mux/2
  Velocity Integrator/3(" theta") -> Mux/3

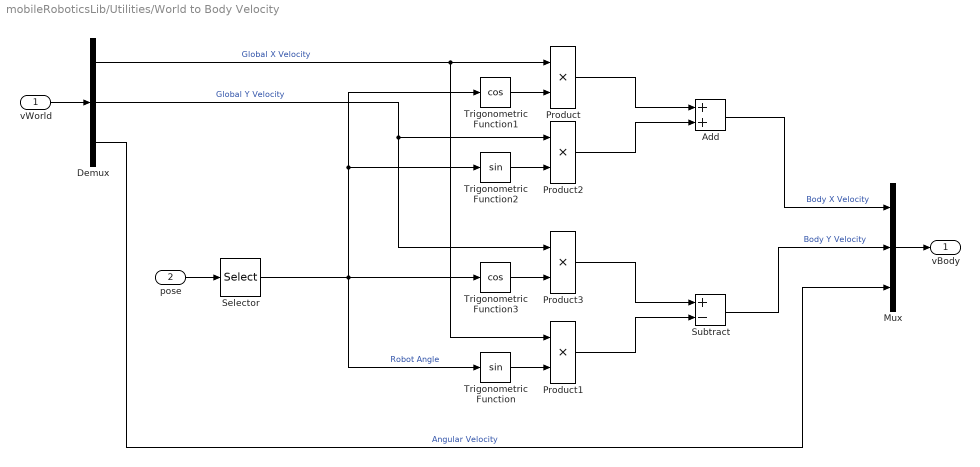
== system mobileRoboticsLib/Utilities/World to Body Velocity ==
  vWorld : Inport
  pose : Inport  Port=2
  Add : Sum
  Demux : Demux  Outputs=3
  Mux : Mux  Inputs=3
  Product{,1..3} (4 alike) : Product
  Selector : Selector  InputPortWidth=3  IndexOptions=Index vector (dialog)  Indices=3  OutputSizes=1
  Subtract : Sum  Inputs=+-
  Trigonometric Function : Trigonometry
  Trigonometric Function1 : Trigonometry  Operator=cos
  Trigonometric Function2 : Trigonometry
  Trigonometric Function3 : Trigonometry  Operator=cos
  vBody : Outport  VectorParamsAs1DForOutWhenUnconnected=off
  wires:
  Trigonometric Function/1 -> Product1/2
  Product1/1 -> Subtract/2
  Product/1 -> Add/1
  Trigonometric Function1/1 -> Product/2
  Demux/1 -> Product/1, Product1/1  "Global X Velocity"
  Selector/1 -> Trigonometric Function/1, Trigonometric Function3/1, Trigonometric Function2/1, Trigonometric Function1/1  "Robot Angle"
  Add/1 -> Mux/1  "Body X Velocity"
  Trigonometric Function2/1 -> Product2/2
  Demux/2 -> Product3/1, Product2/1  "Global Y Velocity"
  Product2/1 -> Add/2
  Trigonometric Function3/1 -> Product3/2
  Product3/1 -> Subtract/1
  Subtract/1 -> Mux/2  "Body Y Velocity"
  vWorld/1 -> Demux/1
  Demux/3 -> Mux/3  "Angular Velocity"
  Mux/1 -> vBody/1
  pose/1 -> Selector/1

== system mobileRoboticsLib/Environments/Multi-Robot Environment/ObjectDetectorParams ==
  Vector Concatenate : Concatenate  NumInputs=3  Mode=Multidimensional array  ConcatenateDimension=2
  objDetParams : Outport
  wires:
  Vector Concatenate/1 -> objDetParams/1
  [slMultiRobotEnv_ObjDet_1] -> Vector Concatenate/1
  [slMultiRobotEnv_ObjDet_2] -> Vector Concatenate/2
  [slMultiRobotEnv_ObjDet_3] -> Vector Concatenate/3

== system mobileRoboticsLib/Environments/Multi-Robot Environment/Poses ==
  Vector Concatenate : Concatenate  NumInputs=3  Mode=Multidimensional array  ConcatenateDimension=2
  poses : Outport
  wires:
  Vector Concatenate/1 -> poses/1
  [slMultiRobotEnv_Pose_1] -> Vector Concatenate/1
  [slMultiRobotEnv_Pose_2] -> Vector Concatenate/2
  [slMultiRobotEnv_Pose_3] -> Vector Concatenate/3

== system mobileRoboticsLib/Environments/Multi-Robot Environment/Ranges ==
  Vector Concatenate : Concatenate  NumInputs=3  Mode=Multidimensional array  ConcatenateDimension=2
  ranges : Outport
  wires:
  Vector Concatenate/1 -> ranges/1
  [slMultiRobotEnv_Ranges_1] -> Vector Concatenate/1
  [slMultiRobotEnv_Ranges_2] -> Vector Concatenate/2
  [slMultiRobotEnv_Ranges_3] -> Vector Concatenate/3

== system mobileRoboticsLib/Environments/Multi-Robot Environment/RobotDetectorParams ==
  Vector Concatenate : Concatenate  NumInputs=3  Mode=Multidimensional array  ConcatenateDimension=2
  robotDetParams : Outport
  wires:
  Vector Concatenate/1 -> robotDetParams/1
  [slMultiRobotEnv_RobotDet_1] -> Vector Concatenate/1
  [slMultiRobotEnv_RobotDet_2] -> Vector Concatenate/2
  [slMultiRobotEnv_RobotDet_3] -> Vector Concatenate/3

== system mobileRoboticsLib/Environments/Multi-Robot Environment/Visuals ==
  Vector Concatenate : Concatenate  NumInputs=3  Mode=Multidimensional array  ConcatenateDimension=2
  visuals : Outport
  wires:
  Vector Concatenate/1 -> visuals/1
  [slMultiRobotEnv_Visuals_1] -> Vector Concatenate/1
  [slMultiRobotEnv_Visuals_2] -> Vector Concatenate/2
  [slMultiRobotEnv_Visuals_3] -> Vector Concatenate/3

== system mobileRoboticsLib/Environments/Multi-Robot Lidar Sensor/Poses ==
  Vector Concatenate : Concatenate  NumInputs=3  Mode=Multidimensional array  ConcatenateDimension=2
  poses : Outport
  wires:
  Vector Concatenate/1 -> poses/1
  [slMultiRobotEnv_Pose_1] -> Vector Concatenate/1
  [slMultiRobotEnv_Pose_2] -> Vector Concatenate/2
  [slMultiRobotEnv_Pose_3] -> Vector Concatenate/3

== system mobileRoboticsLib/Environments/Multi-Robot Lidar Sensor/Visuals ==
  Selector : Selector  NumberOfDimensions=2  InputPortWidth=3  IndexOptions=Index vector (dialog),Select all  Indices=1,1  OutputSizes=1,1
  Vector Concatenate : Concatenate  NumInputs=3  Mode=Multidimensional array  ConcatenateDimension=2
  visuals : Outport
  wires:
  Vector Concatenate/1 -> Selector/1
  Selector/1 -> visuals/1
  [slMultiRobotEnv_Visuals_1] -> Vector Concatenate/1
  [slMultiRobotEnv_Visuals_2] -> Vector Concatenate/2
  [slMultiRobotEnv_Visuals_3] -> Vector Concatenate/3

== system mobileRoboticsLib/Environments/Robot Detector/Poses ==
  Vector Concatenate : Concatenate  NumInputs=3  Mode=Multidimensional array  ConcatenateDimension=2
  poses : Outport
  wires:
  Vector Concatenate/1 -> poses/1
  [slMultiRobotEnv_Pose_1] -> Vector Concatenate/1
  [slMultiRobotEnv_Pose_2] -> Vector Concatenate/2
  [slMultiRobotEnv_Pose_3] -> Vector Concatenate/3
